simulink model "Read_IMU_Height_Kalman_LP_HP_Raw"  (R2019a)
settings: Solver=ode2  StartTime=0.0  StopTime=inf  FixedStep=0.001  RelTol=1e-3  EnableMultiTasking=on
model workspace (MAT data in the model file):
  target_system = 1
undefined symbols (not defined in the file or in its folder): HIL, qc_get_step_size
libraries: quarc_library x6, simulink x1
settings Model: SimulationMode=external  ExtModeTrigDuration=10000  Creator=dmadill  LastModifiedBy=user
settings SolverCC: PositivePriorityOrder=on
settings DataIOCC: LimitDataPoints=on  SaveFormat=Array  ReturnWorkspaceOutputs=off
settings OptimizationCC: LifeSpan=inf
settings DebuggingCC: SolverPrmCheckMsg=warning  SFUnexpectedBacktrackingDiag=warning  SFNoUnconditionalDefaultTransitionDiag=warning  SFExecutionAtInitializationDiag=none  ArithmeticOperatorsInVariantConditions=warning
settings HardwareCC: ProdBitPerLong=64  ProdLargestAtomicFloat=None  ProdHWDeviceType=Intel->x86-64
settings ModelReferenceCC: PropagateSignalLabelsOutOfModel=off
settings SFSimCC: SimUseLocalCustomCode=off
settings RTWCC: SystemTargetFile=quarc_linux_x64.tlc  TemplateMakefile=quarc_linux_x64_tmf  Description=QUARC Linux x64 Target  RTWUseLocalCustomCode=off
settings CodeAppCC: StateflowObjectComments=on
settings STFCustomTargetCC: TargetLibSuffix=.a  TargetPreCompLibLocation=C:\PROGRA~3\QUARC\lib\2019a\LINUX_~1\release  ConcurrentExecutionCompliant=on  SystemTargetFile=quarc_linux_x64.tlc
settings GRTTargetCC: TargetLibSuffix=.a  TargetPreCompLibLocation=C:\PROGRA~3\QUARC\lib\2019a\LINUX_~1\release  TargetLangStandard=C89/C90 (ANSI)  ParMdlRefBuildCompliant=off  CompOptLevelCompliant=off  CombineOutputUpdateFcns=off  MatFileLogging=off  CPPClassGenCompliant=off  GRTInterface=on  UseToolchainInfoCompliant=off  ExtMode=on  ExtModeMexFile=quarc_comm  ExtModeMexArgs='-w -d /tmp -uri %u', 'tcpip://192.168.2.52:17001?retries=10', 'tcpip://192.168.2.52:17000'
settings ConfigComp: CovMetricSettings=dw  CovHtmlReporting=on  CovSaveCumulativeToWorkspaceVar=on  CovSaveSingleToWorkspaceVar=on  CovExternalEMLEnable=off  CovSFcnEnable=off

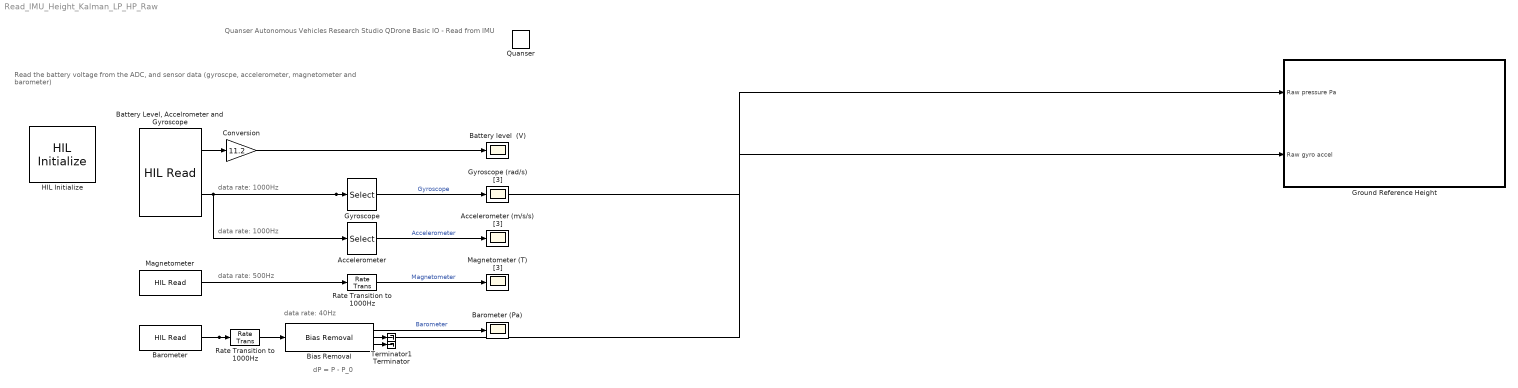
== system Read_IMU_Height_Kalman_LP_HP_Raw ==
  note: Quanser Autonomous Vehicles Research Studio
      | QDrone Basic IO - Read from IMU
  note: Read the battery voltage from the ADC, and sensor data (gyroscpe, accelerometer, magnetometer and barometer)
  note: data rate: 40Hz
  note: dP = P - P_0
  note: data rate: 500Hz
  note: data rate: 1000Hz
  note: data rate: 1000Hz
  Accelerometer : Selector  InputPortWidth=6  IndexOptions=Index vector (dialog)  Indices=[4:6]  OutputSizes=1
  Accelerometer (m/s/s) [3] : Scope
  Barometer : quarc_library/Data Acquisition/Generic/Immediate I//O/HIL Read  Priority=1  object_name=HIL-1  analog_channels=[]  encoder_channels=[]  digital_channels=[]  other_channels=[9000]  sample_time=qc_get_step_size*25  active=on  vector_output=on  data_type_mode=Inherit via back propagation  encoder_data_type=double  digital_data_type=boolean
      settings: SourceProductName=The database C:\Users\user\AppData\Roaming\MathWorks\MATLAB\R2017a\slblocks_master.db is locked, or a table in the database is locked. (database is locked)
  Barometer (Pa) : Scope
  "Battery Level, Accelrometer and Gyroscope" : quarc_library/Data Acquisition/Generic/Immediate I//O/HIL Read  Priority=1  object_name=HIL-1  analog_channels=[4]  encoder_channels=[]  digital_channels=[]  other_channels=[3000:3002 4000:4002]  sample_time=qc_get_step_size  active=on  vector_output=on  data_type_mode=Inherit via back propagation  encoder_data_type=double  digital_data_type=boolean
      settings: SourceProductName=The database C:\Users\user\AppData\Roaming\MathWorks\MATLAB\R2017a\slblocks_master.db is locked, or a table in the database is locked. (database is locked)
  Battery level  (V) : Scope
  Bias Removal : quarc_library/Discrete/Bias Removal  start_time=0  end_time=2  switch_id=X  sample_time=qc_get_step_size
      settings: SourceProductName=QUARC Targets
  Conversion : Gain  Gain=11.2
  Ground Reference Height : Subsystem
  Gyroscope : Selector  InputPortWidth=6  IndexOptions=Index vector (dialog)  Indices=[1:3]  OutputSizes=1
  Gyroscope (rad/s) [3] : Scope
  HIL Initialize : quarc_library/Data Acquisition/Generic/Configuration/HIL Initialize  object_name=HIL-1  board_type=qdrone  board_number=0  board_options=gyro_fs=2000;gyro_rate=1000;gyro_os=4;accel_fs=16;accel_rate=400;accel_os=4;baro_os=4096  exclusive=off  active=on  hardware_clocks=[]  clock_modes=[]  initial_clock_frequencies=[]  set_clock_params_at_start=off  set_clock_params_at_switch_in=off  set_clock_frequencies_at_start=off  set_clock_frequencies_at_switch_in=off  analog_input_channels=[0:4]  analog_input_configurations=[]  analog_input_maximums=[3.3]  analog_input_minimums=[0]  set_analog_input_params_at_start=off  set_analog_input_params_at_switch_in=off  analog_output_channels=[]  analog_output_maximums=[]  analog_output_minimums=[]  initial_analog_outputs=[]  final_analog_outputs=[]  watchdog_analog_outputs=[]  set_analog_output_params_at_start=off  set_analog_output_params_at_switch_in=off  set_analog_outputs_at_start=off  set_analog_outputs_at_switch_in=off  set_analog_outputs_at_terminate=off  set_analog_outputs_at_switch_out=off  set_analog_outputs_on_watchdog=off  digital_input_channels=[]  digital_output_channels=[]  digital_output_configuration=[]  initial_digital_outputs=[0]  final_digital_outputs=[0]  watchdog_digital_outputs=[]  set_digital_output_params_at_start=off  set_digital_output_params_at_switch_in=off  set_digital_outputs_at_start=off  set_digital_outputs_at_switch_in=off  set_digital_outputs_at_terminate=off  set_digital_outputs_at_switch_out=off  set_digital_outputs_on_watchdog=off  encoder_channels=[]  quadrature=[4]  encoder_filter_frequency=50e6/1  initial_encoder_counts=[0]  set_encoder_params_at_start=off  set_encoder_params_at_switch_in=off  set_encoder_counts_at_start=off  set_encoder_counts_at_switch_in=off  pwm_channels=[]  pwm_modes=[4]  pwm_frequency=2000  pwm_configuration=[0]  pwm_alignment=[0]  pwm_polarity=[1]  pwm_leading_deadband=[]  pwm_trailing_deadband=[]  initial_pwm_outputs=[0]  final_pwm_outputs=[0]  watchdog_pwm_outputs=[0]  set_pwm_params_at_start=off  set_pwm_params_at_switch_in=off  set_pwm_outputs_at_start=off  set_pwm_outputs_at_switch_in=off  set_pwm_outputs_at_terminate=off  set_pwm_outputs_at_switch_out=off  set_pwm_outputs_on_watchdog=off  other_output_channels=[]  initial_other_outputs=[]  final_other_outputs=[]  watchdog_other_outputs=[]  set_other_outputs_at_start=off  set_other_outputs_at_switch_in=off  set_other_outputs_at_terminate=off  set_other_outputs_at_switch_out=off  set_other_outputs_on_watchdog=off
      settings: SourceProductName=The database C:\Users\user\AppData\Roaming\MathWorks\MATLAB\R2017a\slblocks_master.db is locked, or a table in the database is locked. (database is locked)
  Magnetometer : quarc_library/Data Acquisition/Generic/Immediate I//O/HIL Read  Priority=1  object_name=HIL-1  analog_channels=[]  encoder_channels=[]  digital_channels=[]  other_channels=[8000:8002]  sample_time=qc_get_step_size*2  active=on  vector_output=on  data_type_mode=Inherit via back propagation  encoder_data_type=double  digital_data_type=boolean
      settings: SourceProductName=The database C:\Users\user\AppData\Roaming\MathWorks\MATLAB\R2017a\slblocks_master.db is locked, or a table in the database is locked. (database is locked)
  Magnetometer (T) [3] : Scope
  Quanser : quarc_library/Logos/Quanser
  Rate Transition to 1000Hz : RateTransition
  Rate Transition to 1000Hz : RateTransition  OutPortSampleTime=qc_get_step_size
  Terminator : Terminator
  Terminator1 : Terminator
  wires:
  Accelerometer/1 -> Accelerometer (m/s/s) [3]/1  "Accelerometer"
  Bias Removal/3 -> Terminator/1
  Gyroscope/1 -> Gyroscope (rad/s) [3]/1  "Gyroscope"
  Barometer/1 -> Rate Transition to 1000Hz/1, Ground Reference Height/1(Raw pressure Pa)
  Bias Removal/1 -> Barometer (Pa)/1  "Barometer"
  "Battery Level, Accelrometer and Gyroscope"/1 -> Conversion/1
  Bias Removal/2 -> Terminator1/1
  Magnetometer/1 -> Rate Transition to 1000Hz/1
  Rate Transition to 1000Hz/1 -> Magnetometer (T) [3]/1  "Magnetometer"
  Conversion/1 -> Battery level  (V)/1
  "Battery Level, Accelrometer and Gyroscope"/2 -> Ground Reference Height/2(Raw gyro accel), Gyroscope/1, Accelerometer/1
  Rate Transition to 1000Hz/1 -> Bias Removal/1

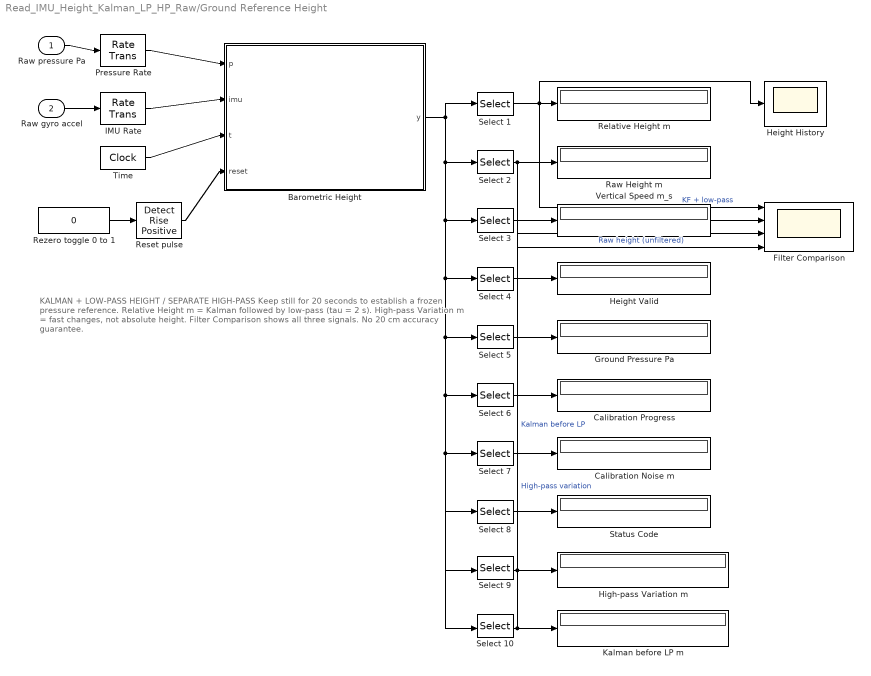
== system Read_IMU_Height_Kalman_LP_HP_Raw/Ground Reference Height ==
  note: KALMAN + LOW-PASS HEIGHT / SEPARATE HIGH-PASS
      | Keep still for 20 seconds to establish a frozen pressure reference.
      | Relative Height m = Kalman followed by low-pass (tau = 2 s).
      | High-pass Variation m = fast changes, not absolute height.
      | Filter Comparison shows all three signals. No 20 cm accuracy guarantee.
  Raw pressure Pa : Inport
  Raw gyro accel : Inport  Port=2
  Barometric Height : MATLAB Function  TreatAsAtomicUnit=on
  Calibration Noise m : Display
  Calibration Progress : Display
  Ground Pressure Pa : Display
  Height History : Scope
  Height Valid : Display
  IMU Rate : RateTransition  OutPortSampleTime=0.025
  Pressure Rate : RateTransition  OutPortSampleTime=0.025
  Raw Height m : Display
  Relative Height m : Display
  Reset pulse : simulink/Logic and Bit Operations/Detect Rise Positive  vinit=0  OutDataTypeStr=boolean
  Rezero toggle 0 to 1 : Constant  Value=0  SampleTime=0.025
  Select 1 : Selector  InputPortWidth=10  IndexOptions=Index vector (dialog)  Indices=1  OutputSizes=1
  Select 2 : Selector  InputPortWidth=10  IndexOptions=Index vector (dialog)  Indices=2  OutputSizes=1
  Select 3 : Selector  InputPortWidth=10  IndexOptions=Index vector (dialog)  Indices=3  OutputSizes=1
  Select 4 : Selector  InputPortWidth=10  IndexOptions=Index vector (dialog)  Indices=4  OutputSizes=1
  Select 5 : Selector  InputPortWidth=10  IndexOptions=Index vector (dialog)  Indices=5  OutputSizes=1
  Select 6 : Selector  InputPortWidth=10  IndexOptions=Index vector (dialog)  Indices=6  OutputSizes=1
  Select 7 : Selector  InputPortWidth=10  IndexOptions=Index vector (dialog)  Indices=7  OutputSizes=1
  Select 8 : Selector  InputPortWidth=10  IndexOptions=Index vector (dialog)  Indices=8  OutputSizes=1
  Status Code : Display
  Time : DigitalClock  SampleTime=0.025
  Vertical Speed m_s : Display
  Select 9 : Selector  InputPortWidth=10  IndexOptions=Index vector (dialog)  Indices=9  OutputSizes=1
  High-pass Variation m : Display
  Select 10 : Selector  InputPortWidth=10  IndexOptions=Index vector (dialog)  Indices=10  OutputSizes=1
  Kalman before LP m : Display
  Filter Comparison : Scope  NumInputPorts=4
  wires:
  Raw pressure Pa/1 -> Pressure Rate/1
  Pressure Rate/1 -> Barometric Height/1(p)
  Raw gyro accel/1 -> IMU Rate/1
  IMU Rate/1 -> Barometric Height/2(imu)
  Time/1 -> Barometric Height/3(t)
  Rezero toggle 0 to 1/1 -> Reset pulse/1
  Reset pulse/1 -> Barometric Height/4(reset)
  Barometric Height/1(y) -> Select 7/1, Select 8/1, Select 6/1, Select 5/1, Select 4/1, Select 3/1, Select 2/1, Select 1/1, Select 9/1, Select 10/1
  Select 1/1 -> Relative Height m/1, Height History/1, Filter Comparison/1  "KF + low-pass"
  Select 2/1 -> Raw Height m/1, Filter Comparison/4  "Raw height (unfiltered)"
  Select 3/1 -> Vertical Speed m_s/1
  Select 4/1 -> Height Valid/1
  Select 5/1 -> Ground Pressure Pa/1
  Select 6/1 -> Calibration Progress/1
  Select 7/1 -> Calibration Noise m/1
  Select 8/1 -> Status Code/1
  Select 9/1 -> High-pass Variation m/1, Filter Comparison/3  "High-pass variation"
  Select 10/1 -> Kalman before LP m/1, Filter Comparison/2  "Kalman before LP"

== matlab function Read_IMU_Height_Kalman_LP_HP_Raw/Ground Reference Height/Barometric Height ==
  data: p input; y output; imu input; t input; reset input
function y=run(p,imu,t,reset)
%#codegen
g=sqrt(sum(imu(1:3).^2));
a=sqrt(sum(imu(4:6).^2));
base=qdrone_baro_height_kalman_smooth(p,t,g,a,reset);
y=qdrone_height_lp_hp_step(base,t,reset);
end

function y = qdrone_baro_height_kalman_smooth(p,t,gyroNorm,accelNorm,reset)
%#codegen
% Stronger smoothing variant: q reduced from 0.25 to 0.025.
% Relative barometric height [m] and vertical speed [m/s], upward positive.
% Smoother output trades off slower tracking. It does not remove barometer drift.
% p: RAW pressure [Pa]; t: time [s]; gyroNorm [rad/s]; accelNorm [m/s^2].
% reset: one-sample pulse. Call once per new barometer sample (0.025 s).
% The calibration helper is embedded below in this block.
% y=[height;raw_height;speed;valid;reference_Pa;progress;noise_m;status].
persistent x P lastT
if isempty(lastT)
    x = zeros(2,1);
    P = eye(2);
    lastT = NaN;
end
% Existing validation and 20-second stationary pressure reference.
y = qdrone_baro_height(p,t,gyroNorm,accelNorm,reset);
if reset || (isfinite(lastT) && isfinite(t) && t < lastT)
    lastT = NaN;
end
if y(4) == 0
    y(1) = NaN;
    y(3) = NaN;
    lastT = NaN;
    return;
end
sigma = max(0.05,y(7)); % Measurement standard deviation [m].
R = sigma^2;
q = 0.025;              % Acceleration spectral density [m^2/s^3].
z = y(2);              % Raw height, before the existing low-pass filter.
if ~isfinite(lastT)
    x = [z;0];
    P = [R 0;0 1];
else
    dt = t-lastT;
    A = [1 dt;0 1];
    Q = q*[dt^3/3 dt^2/2;dt^2/2 dt];
    % Predict state [height; vertical speed].
    xp = A*x;
    Pp = A*P*A' + Q;
    % Correct using height measurement, H=[1 0].
    K = Pp(:,1)/(Pp(1,1)+R);
    x = xp + K*(z-xp(1));
    % Joseph covariance update.
    J = eye(2)-K*[1 0];
    P = J*Pp*J' + K*R*K';
    P = (P+P')/2;
end
lastT = t;
y(1) = x(1);
y(3) = x(2);
end

function y=qdrone_baro_height(p,t,gyroNorm,accelNorm,reset)
%#codegen
% BAROMETRIC relative height; no direct measurement of distance to the floor.
% Average 20 seconds of stationary raw pressure, then FREEZE p0.
% Only explicit reset or a new/rewound model clock can clear the reference.
% y=[filtered_m raw_m vertical_m_s valid reference_Pa progress noise_m status].
% status: 0 calibrating,1 valid,2 invalid pressure,3 moving during calibration,
% 4 time gap/rewind,5 pressure jump,6 noisy calibration rejected.
persistent p0 count pressureMean pressureM2 beginTime lastTick lastGood lastP filtered speed noise
if isempty(count)
 p0=NaN;count=0;pressureMean=0;pressureM2=0;beginTime=NaN;lastTick=NaN;
 lastGood=NaN;lastP=NaN;filtered=NaN;speed=0;noise=NaN;
end
rewind=isfinite(lastTick)&&isfinite(t)&&t<lastTick;
if reset || rewind
 p0=NaN;count=0;pressureMean=0;pressureM2=0;beginTime=NaN;lastTick=NaN;
 lastGood=NaN;lastP=NaN;filtered=NaN;speed=0;noise=NaN;
end
y=[NaN;NaN;NaN;0;p0;0;noise;0];
if ~isfinite(t)||(isfinite(lastTick)&&t<=lastTick),y(8)=4;return;end
previousTick=lastTick;lastTick=t;
if ~isfinite(p)||p<50000||p>110000
 if ~isfinite(p0),count=0;pressureMean=0;pressureM2=0;beginTime=NaN;end
 filtered=NaN;y(8)=2;return;
end
if isfinite(previousTick)&&t-previousTick>0.5
 filtered=NaN;lastGood=NaN;
 if ~isfinite(p0),count=0;pressureMean=0;pressureM2=0;beginTime=NaN;end
 y(8)=4;return;
end
if ~isfinite(p0)
 stationary=isfinite(gyroNorm)&&isfinite(accelNorm)&&gyroNorm<0.05&&accelNorm>8.8&&accelNorm<10.8;
 if ~stationary
  count=0;pressureMean=0;pressureM2=0;beginTime=NaN;y(8)=3;return;
 end
 if count==0,beginTime=t;end
 % Welford accumulation uses the ENTIRE calibration interval, not a capped array.
 count=count+1;delta=p-pressureMean;pressureMean=pressureMean+delta/count;
 pressureM2=pressureM2+delta*(p-pressureMean);
 elapsed=t-beginTime;y(6)=min(1,elapsed/20);
 if elapsed<20||count<200,return;end
 sigma=sqrt(max(0,pressureM2/max(1,count-1)));
 if sigma>4
  count=0;pressureMean=0;pressureM2=0;beginTime=NaN;y(6)=0;y(8)=6;return;
 end
 p0=pressureMean;noise=(44330/5.25588)*sigma/p0;
 filtered=0;speed=0;lastGood=t;lastP=p;
 raw=44330*(1-(p/p0)^(1/5.25588));
 y=[0;raw;0;1;p0;1;noise;1];return;
end
% From here p0 is read-only: no autozero and no adaptation at a held height.
raw=44330*(1-(p/p0)^(1/5.25588));
if isfinite(lastGood)&&t-lastGood<=0.5&&abs(p-lastP)>200
 filtered=NaN;y(5)=p0;y(8)=5;return;
end
if ~isfinite(filtered)||~isfinite(lastGood)||t-lastGood>0.5
 filtered=raw;speed=0;
else
 dt=t-lastGood;old=filtered;alpha=1-exp(-dt/0.5);
 filtered=filtered+alpha*(raw-filtered);
 speed=speed+(1-exp(-dt/1.0))*((filtered-old)/dt-speed);
end
lastGood=t;lastP=p;
y=[filtered;raw;speed;1;p0;1;noise;1];
end

function y = qdrone_height_lp_hp_step(base,t,reset)
%#codegen
% Post-filter the 8-element calibrated Kalman output.
% y(1): Kalman + low-pass height [m]; y(3): its discrete slope [m/s].
% y(9): high-pass variation of RAW height [m], not absolute height.
% y(10): Kalman height before low-pass [m]. Other fields keep their meaning.
% Filters reset on unavailable data and reinitialize on valid recovery.
persistent lowHeight highVariation previousRaw lastT
if isempty(lastT)
    lowHeight = 0;
    highVariation = 0;
    previousRaw = 0;
    lastT = NaN;
end
y = [base;NaN;NaN];
if reset
    lastT = NaN;
end
if base(4)==0 || ~isfinite(base(1)) || ~isfinite(base(2)) || ~isfinite(t)
    lastT = NaN;
    y(1) = NaN; y(3) = NaN; y(4) = 0;
    return;
end

tauLP = 2.0; % Low-pass time constant [s], cutoff about 0.080 Hz.
tauHP = 2.0; % High-pass time constant [s], cutoff about 0.080 Hz.
if ~isfinite(lastT) || t<lastT || t-lastT>0.5
    lowHeight = base(1);
    highVariation = 0;
    speed = 0;
elseif t==lastT
    lastT = NaN;
    y(1) = NaN; y(3) = NaN; y(4) = 0; y(8) = 4;
    return;
else
    dt = t-lastT;
    alpha = dt/(tauLP+dt);
    previousLow = lowHeight;
    lowHeight = lowHeight+alpha*(base(1)-lowHeight);
    speed = (lowHeight-previousLow)/dt;
    beta = tauHP/(tauHP+dt);
    highVariation = beta*(highVariation+base(2)-previousRaw);
end
lastT = t;
previousRaw = base(2);
y(1) = lowHeight;
y(3) = speed;
y(9) = highVariation;
y(10) = base(1);
end
